simulink model "AXU5EV_R5_Reference"  (R2026b)
settings: Solver=FixedStepDiscrete  StopTime=0.1  FixedStep=Ts_ACR
undefined symbols (not defined in the file): Hold_Ticks, Id_Init_Step, Id_Init_Target, Id_Release_Ramp_Ticks, Iq_fric_run, Iq_fric_start, Iq_int_limit, Kaw_d, Kaw_q, Kaw_s, Ki_ACR, Ki_ASR, Kp_ACR, Kp_ASR, Kp_pos, PMLSM_Ld_H, PMLSM_Lq_H, PMLSM_psi_f_Wb, Pos_deadband, Ramp_Ticks, Speed_loop_Iq_Limit, T_pwm, Tau_e_mm, theta_align_const, Ts, Ts_ACR, Ts_ASR, Udc, v_ff_eps, v_over_eps, V_pos_max_mmps, v_ref_max, v_ref_set_step_dn, v_ref_set_step_up, v_ref_zero_eps, v_stick_off, v_stick_on
libraries: simulink x7, mcbeeMathTransformLib x2
settings Model: Creator=lww  LastModifiedBy=lww
settings OptimizationCC: DefaultParameterBehavior=Inlined  DifferentSizesBufferReuse=on  EfficientTunableParamExpr=on  EnhancedBackFolding=on  OptimizationCustomize=off  OptimizeBlockOrder=speed  PassReuseOutputArgsAs=Individual arguments  RemoveInternalMemoryZeroInit=on  RemoveRootLevelIOMemoryZeroInit=on
settings DebuggingCC: ParameterTunabilityLossMsg=error
settings SFSimCC: MATLABDynamicMemAlloc=off
settings RTWCC: DataTypeReplacement=CDataTypesFixedWidth  Description=Embedded Coder  GenCodeOnly=on  SystemTargetFile=ert.tlc  TemplateMakefile=ert_default_tmf
settings CodeAppCC: ForceParamTrailComments=on  IgnoreCustomStorageClasses=off  InsertBlockDesc=on  OperatorAnnotations=on  SFDataObjDesc=on  SimulinkDataObjDesc=on
settings ERTTargetCC: CombineSignalStateStructs=on  GenerateSampleERTMain=on  MaxIdInt16=INT16_MAX  MaxIdInt32=INT32_MAX  MaxIdInt64=INT64_MAX  MaxIdInt8=INT8_MAX  MaxIdUint16=UINT16_MAX  MaxIdUint32=UINT32_MAX  MaxIdUint64=UINT64_MAX  MaxIdUint8=UINT8_MAX  MinIdInt16=INT16_MIN  MinIdInt32=INT32_MIN  MinIdInt64=INT64_MIN  MinIdInt8=INT8_MIN

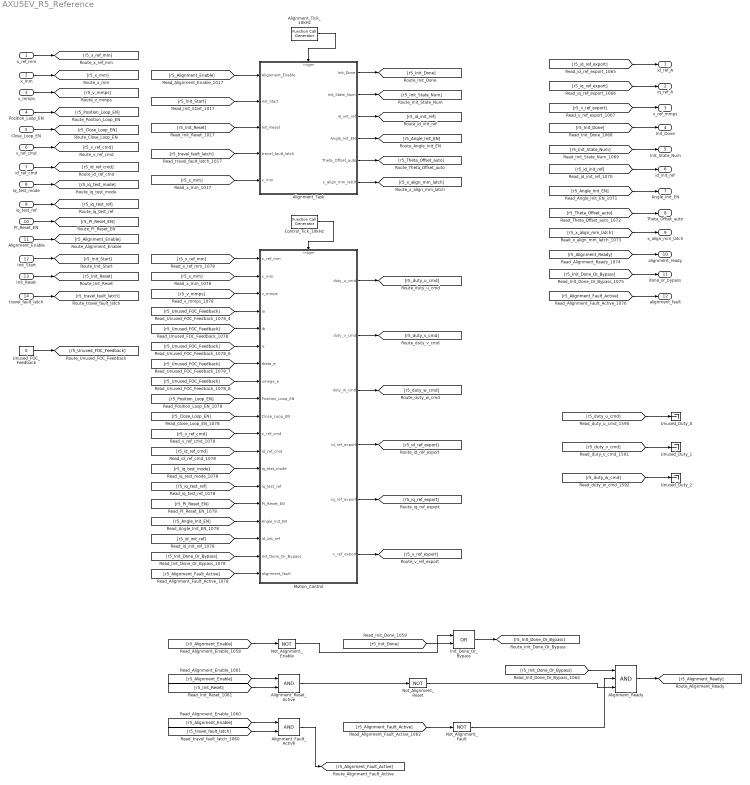
== system AXU5EV_R5_Reference ==
  x_ref_mm : Inport  OutDataTypeStr=double  SampleTime=Ts_ACR
  x_mm : Inport  Port=2  OutDataTypeStr=double  SampleTime=Ts_ACR
  v_mmps : Inport  Port=3  OutDataTypeStr=double  SampleTime=Ts_ACR
  Position_Loop_EN : Inport  Port=4  OutDataTypeStr=double  SampleTime=Ts_ACR
  Close_Loop_EN : Inport  Port=5  OutDataTypeStr=double  SampleTime=Ts_ACR
  v_ref_cmd : Inport  Port=6  OutDataTypeStr=double  SampleTime=Ts_ACR
  id_ref_cmd : Inport  Port=7  OutDataTypeStr=double  SampleTime=Ts_ACR
  iq_test_mode : Inport  Port=8  OutDataTypeStr=double  SampleTime=Ts_ACR
  iq_test_ref : Inport  Port=9  OutDataTypeStr=double  SampleTime=Ts_ACR
  PI_Reset_EN : Inport  Port=10  OutDataTypeStr=double  SampleTime=Ts_ACR
  Alignment_Enable : Inport  Port=11  OutDataTypeStr=double  SampleTime=Ts_ACR
  Init_Start : Inport  Port=12  OutDataTypeStr=double  SampleTime=Ts_ACR
  Init_Reset : Inport  Port=13  OutDataTypeStr=double  SampleTime=Ts_ACR
  travel_fault_latch : Inport  Port=14  OutDataTypeStr=double  SampleTime=Ts_ACR
  Alignment_Fault_Active : Logic  IconShape=distinctive  AllPortsSameDT=off  OutDataTypeStr=boolean
  Alignment_Ready : Logic  Inputs=3  IconShape=distinctive  AllPortsSameDT=off  OutDataTypeStr=boolean
  Alignment_Reset_Active : Logic  IconShape=distinctive  AllPortsSameDT=off  OutDataTypeStr=boolean
  Alignment_Task : Subsystem
  Alignment_Tick_10kHz : FunctionCallGenerator  Priority=-100  SampleTime=Ts
  Control_Tick_10kHz : FunctionCallGenerator  Priority=100  SampleTime=Ts
  Init_Done_Or_Bypass : Logic  Operator=OR  IconShape=distinctive  AllPortsSameDT=off  OutDataTypeStr=boolean
  Motion_Control : Subsystem
  Not_Alignment_Enable : Logic  Operator=NOT  IconShape=distinctive  AllPortsSameDT=off  OutDataTypeStr=boolean
  Not_Alignment_Fault : Logic  Operator=NOT  IconShape=distinctive  AllPortsSameDT=off  OutDataTypeStr=boolean
  Not_Alignment_Reset : Logic  Operator=NOT  IconShape=distinctive  AllPortsSameDT=off  OutDataTypeStr=boolean
  Unused_Duty_0 : Terminator
  Unused_Duty_1 : Terminator
  Unused_Duty_2 : Terminator
  Unused_FOC_Feedback : Constant  Value=0
  id_ref_A : Outport
  iq_ref_A : Outport  Port=2
  v_ref_mmps : Outport  Port=3
  Init_Done : Outport  Port=4
  Init_State_Num : Outport  Port=5
  id_init_ref : Outport  Port=6
  Angle_Init_EN : Outport  Port=7
  Theta_Offset_auto : Outport  Port=8
  x_align_mm_latch : Outport  Port=9
  alignment_ready : Outport  Port=10
  done_or_bypass : Outport  Port=11
  alignment_fault : Outport  Port=12
  wires:
  Unused_FOC_Feedback/1 -> [r5_Unused_FOC_Feedback]
  [r5_Unused_FOC_Feedback] -> Motion_Control/5(ib)
  Alignment_Ready/1 -> [r5_Alignment_Ready]
  [r5_Alignment_Ready] -> alignment_ready/1
  Alignment_Fault_Active/1 -> [r5_Alignment_Fault_Active]
  [r5_Alignment_Fault_Active] -> Not_Alignment_Fault/1
  [r5_Alignment_Fault_Active] -> alignment_fault/1
  [r5_Alignment_Fault_Active] -> Motion_Control/19(alignment_fault)
  Init_Done_Or_Bypass/1 -> [r5_Init_Done_Or_Bypass]
  [r5_Init_Done_Or_Bypass] -> Motion_Control/18(Init_Done_Or_Bypass)
  [r5_Init_Done_Or_Bypass] -> done_or_bypass/1
  [r5_Init_Done_Or_Bypass] -> Alignment_Ready/1
  Motion_Control/6(v_ref_export) -> [r5_v_ref_export]
  [r5_v_ref_export] -> v_ref_mmps/1
  Motion_Control/5(iq_ref_export) -> [r5_iq_ref_export]
  [r5_iq_ref_export] -> iq_ref_A/1
  Motion_Control/4(id_ref_export) -> [r5_id_ref_export]
  [r5_id_ref_export] -> id_ref_A/1
  Motion_Control/3(duty_w_cmd) -> [r5_duty_w_cmd]
  [r5_duty_w_cmd] -> Unused_Duty_2/1
  Motion_Control/2(duty_v_cmd) -> [r5_duty_v_cmd]
  [r5_duty_v_cmd] -> Unused_Duty_1/1
  Motion_Control/1(duty_u_cmd) -> [r5_duty_u_cmd]
  [r5_duty_u_cmd] -> Unused_Duty_0/1
  Alignment_Task/6(x_align_mm_latch) -> [r5_x_align_mm_latch]
  [r5_x_align_mm_latch] -> x_align_mm_latch/1
  Alignment_Task/5(Theta_Offset_auto) -> [r5_Theta_Offset_auto]
  [r5_Theta_Offset_auto] -> Theta_Offset_auto/1
  Alignment_Task/4(Angle_Init_EN) -> [r5_Angle_Init_EN]
  [r5_Angle_Init_EN] -> Angle_Init_EN/1
  [r5_Angle_Init_EN] -> Motion_Control/16(Angle_Init_EN)
  Alignment_Task/3(id_init_ref) -> [r5_id_init_ref]
  [r5_id_init_ref] -> id_init_ref/1
  [r5_id_init_ref] -> Motion_Control/17(id_init_ref)
  Alignment_Task/2(Init_State_Num) -> [r5_Init_State_Num]
  [r5_Init_State_Num] -> Init_State_Num/1
  Alignment_Task/1(Init_Done) -> [r5_Init_Done]
  [r5_Init_Done] -> Init_Done_Or_Bypass/2
  [r5_Init_Done] -> Init_Done/1
  travel_fault_latch/1 -> [r5_travel_fault_latch]
  [r5_travel_fault_latch] -> Alignment_Fault_Active/2
  [r5_travel_fault_latch] -> Alignment_Task/4(travel_fault_latch)
  Init_Reset/1 -> [r5_Init_Reset]
  [r5_Init_Reset] -> Alignment_Task/3(Init_Reset)
  [r5_Init_Reset] -> Alignment_Reset_Active/2
  Init_Start/1 -> [r5_Init_Start]
  [r5_Init_Start] -> Alignment_Task/2(Init_Start)
  Alignment_Enable/1 -> [r5_Alignment_Enable]
  [r5_Alignment_Enable] -> Alignment_Fault_Active/1
  [r5_Alignment_Enable] -> Not_Alignment_Enable/1
  [r5_Alignment_Enable] -> Alignment_Reset_Active/1
  [r5_Alignment_Enable] -> Alignment_Task/1(Alignment_Enable)
  PI_Reset_EN/1 -> [r5_PI_Reset_EN]
  [r5_PI_Reset_EN] -> Motion_Control/15(PI_Reset_EN)
  iq_test_ref/1 -> [r5_iq_test_ref]
  [r5_iq_test_ref] -> Motion_Control/14(iq_test_ref)
  iq_test_mode/1 -> [r5_iq_test_mode]
  [r5_iq_test_mode] -> Motion_Control/13(iq_test_mode)
  id_ref_cmd/1 -> [r5_id_ref_cmd]
  [r5_id_ref_cmd] -> Motion_Control/12(id_ref_cmd)
  v_ref_cmd/1 -> [r5_v_ref_cmd]
  [r5_v_ref_cmd] -> Motion_Control/11(v_ref_cmd)
  Close_Loop_EN/1 -> [r5_Close_Loop_EN]
  [r5_Close_Loop_EN] -> Motion_Control/10(Close_Loop_EN)
  Position_Loop_EN/1 -> [r5_Position_Loop_EN]
  [r5_Position_Loop_EN] -> Motion_Control/9(Position_Loop_EN)
  v_mmps/1 -> [r5_v_mmps]
  [r5_v_mmps] -> Motion_Control/3(v_mmps)
  x_mm/1 -> [r5_x_mm]
  [r5_x_mm] -> Motion_Control/2(x_mm)
  [r5_x_mm] -> Alignment_Task/5(x_mm)
  x_ref_mm/1 -> [r5_x_ref_mm]
  [r5_x_ref_mm] -> Motion_Control/1(x_ref_mm)
  Not_Alignment_Fault/1 -> Alignment_Ready/2
  Alignment_Tick_10kHz/1 -> Alignment_Task/Trigger
  Control_Tick_10kHz/1 -> Motion_Control/Trigger
  Alignment_Reset_Active/1 -> Not_Alignment_Reset/1
  Not_Alignment_Enable/1 -> Init_Done_Or_Bypass/1
  Not_Alignment_Reset/1 -> Alignment_Ready/3
  [r5_Unused_FOC_Feedback] -> Motion_Control/8(omega_e)
  [r5_Unused_FOC_Feedback] -> Motion_Control/7(theta_e)
  [r5_Unused_FOC_Feedback] -> Motion_Control/6(ic)
  [r5_Unused_FOC_Feedback] -> Motion_Control/4(ia)

== system AXU5EV_R5_Reference/Alignment_Task ==
  Alignment_Enable : Inport
  Init_Start : Inport  Port=2
  Init_Reset : Inport  Port=3
  travel_fault_latch : Inport  Port=4
  x_mm : Inport  Port=5
  Tick : TriggerPort  TriggerType=function-call  VariantControl=(inherit)
  Enabled_Original_MIL : Subsystem
  Init_Done : Outport
  Init_State_Num : Outport  Port=2
  id_init_ref : Outport  Port=3
  Angle_Init_EN : Outport  Port=4
  Theta_Offset_auto : Outport  Port=5
  x_align_mm_latch : Outport  Port=6
  wires:
  Enabled_Original_MIL/6(x_align_mm_latch) -> x_align_mm_latch/1
  Enabled_Original_MIL/5(Theta_Offset_auto) -> Theta_Offset_auto/1
  Enabled_Original_MIL/4(Angle_Init_EN) -> Angle_Init_EN/1
  Enabled_Original_MIL/1(Init_Done) -> Init_Done/1
  x_mm/1 -> Enabled_Original_MIL/4(x_mm)
  travel_fault_latch/1 -> Enabled_Original_MIL/3(travel_fault_latch)
  Init_Reset/1 -> Enabled_Original_MIL/2(Init_Reset)
  Enabled_Original_MIL/3(id_init_ref) -> id_init_ref/1
  Init_Start/1 -> Enabled_Original_MIL/1(Init_Start)
  Enabled_Original_MIL/2(Init_State_Num) -> Init_State_Num/1
  Alignment_Enable/1 -> Enabled_Original_MIL/Enable

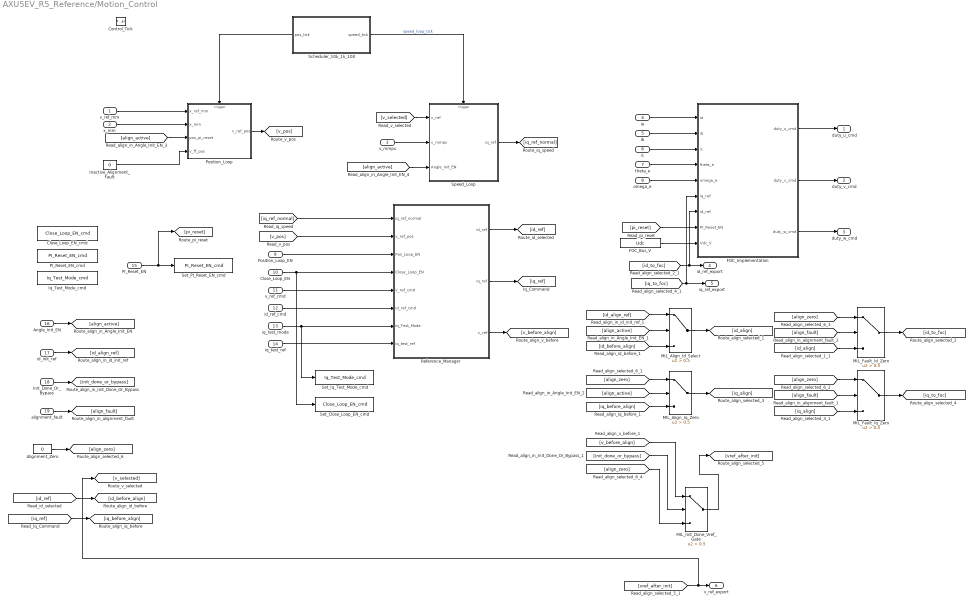
== system AXU5EV_R5_Reference/Motion_Control ==
  x_ref_mm : Inport
  x_mm : Inport  Port=2
  v_mmps : Inport  Port=3
  ia : Inport  Port=4
  ib : Inport  Port=5
  ic : Inport  Port=6
  theta_e : Inport  Port=7
  omega_e : Inport  Port=8
  Position_Loop_EN : Inport  Port=9
  Close_Loop_EN : Inport  Port=10
  v_ref_cmd : Inport  Port=11
  id_ref_cmd : Inport  Port=12
  iq_test_mode : Inport  Port=13
  iq_test_ref : Inport  Port=14
  PI_Reset_EN : Inport  Port=15
  Angle_Init_EN : Inport  Port=16
  id_init_ref : Inport  Port=17
  Init_Done_Or_Bypass : Inport  Port=18
  alignment_fault : Inport  Port=19
  Control_Tick : TriggerPort  TriggerType=function-call  VariantControl=(inherit)  PortDimensions=1
  Alignment_Zero : Constant  Value=0
  Close_Loop_EN_cmd : DataStoreMemory  DataStoreName=Close_Loop_EN_cmd  WriteAfterWriteMsg=warning  InitialValue=1  ShowAdditionalParam=off
  FOC_Bus_V : Constant  Value=Udc  SampleTime=-1
  FOC_Implementation : Subsystem  Variant=on  EmptyChoice=on
  Inactive_Alignment_Fault : Constant  Value=0
  Iq_Test_Mode_cmd : DataStoreMemory  DataStoreName=Iq_Test_Mode_cmd  WriteAfterWriteMsg=warning  ShowAdditionalParam=off
  MIL_Align_Id_Select : Switch  Criteria=u2 > Threshold  Threshold=0.5  SaturateOnIntegerOverflow=off  InputSameDT=off
  MIL_Align_Iq_Zero : Switch  Criteria=u2 > Threshold  Threshold=0.5  SaturateOnIntegerOverflow=off  InputSameDT=off
  MIL_Fault_Id_Zero : Switch  Criteria=u2 > Threshold  Threshold=0.5  SaturateOnIntegerOverflow=off  InputSameDT=off
  MIL_Fault_Iq_Zero : Switch  Criteria=u2 > Threshold  Threshold=0.5  SaturateOnIntegerOverflow=off  InputSameDT=off
  MIL_Init_Done_Vref_Gate : Switch  Criteria=u2 > Threshold  Threshold=0.5  SaturateOnIntegerOverflow=off  InputSameDT=off
  PI_Reset_EN_cmd : DataStoreMemory  DataStoreName=PI_Reset_EN_cmd  WriteAfterWriteMsg=warning  ShowAdditionalParam=off
  Position_Loop : Subsystem  TreatAsAtomicUnit=on
  Reference_Manager : Subsystem
  Scheduler_10k_1k_100 : Subsystem
      settings: PortSchema="{\"entries\":[{\"content\":{\"sides\":[{\"content\":{\"connectorIds\":[\"Out2\"]},\"type\":\"ConnectorPlacement.EquallySpacedRectSide\",\"uuid\":\"7a2cd2ad-1b6d-4ced-b4c0-dea2e76e4441\"},{\"content\":{\"connectorIds\":[\"Out1\"],\"side\":\"RIGHT\"},\"type\":\"ConnectorPlacement.EquallySpacedRectSide\",\"uuid\":\"f7db3b94-1126-4089-83bd-8e57d20e6fd7\"},{\"content\":{\"side\":\"TOP\"},\"type\":\"ConnectorPlacement.EquallySpacedRectSide\",\"uuid\":\"9153f6b5-22af-48be-92c0-68be43f93648\"}]},\"type\":\"ConnectorPlacement.EquallySpacedConnector\",\"uuid\":\"029fb485-bddc-4cd2-9c64-7547c8dffd2b\"}],\"packageUris\":[\"http://schema.mathworks.com/mf0/Connector/R2020b\"],\"version\":\"1.0\"}"
  Set_Close_Loop_EN_cmd : DataStoreWrite  Priority=-10  DataStoreName=Close_Loop_EN_cmd  IndexOptions=Index vector (dialog)  Indices=1  OutputSizes=1
  Set_Iq_Test_Mode_cmd : DataStoreWrite  Priority=-10  DataStoreName=Iq_Test_Mode_cmd  IndexOptions=Index vector (dialog)  Indices=1  OutputSizes=1
  Set_PI_Reset_EN_cmd : DataStoreWrite  Priority=-10  DataStoreName=PI_Reset_EN_cmd  IndexOptions=Index vector (dialog)  Indices=1  OutputSizes=1
  Speed_Loop : Subsystem  TreatAsAtomicUnit=on
  duty_u_cmd : Outport
  duty_v_cmd : Outport  Port=2
  duty_w_cmd : Outport  Port=3
  id_ref_export : Outport  Port=4
  iq_ref_export : Outport  Port=5
  v_ref_export : Outport  Port=6
  wires:
  FOC_Bus_V/1 -> FOC_Implementation/9(Vdc_V)
  FOC_Implementation/3(duty_w_cmd) -> duty_w_cmd/1
  FOC_Implementation/2(duty_v_cmd) -> duty_v_cmd/1
  FOC_Implementation/1(duty_u_cmd) -> duty_u_cmd/1
  [pi_reset] -> FOC_Implementation/8(PI_Reset_EN)
  omega_e/1 -> FOC_Implementation/5(omega_e)
  theta_e/1 -> FOC_Implementation/4(theta_e)
  ic/1 -> FOC_Implementation/3(ic)
  ib/1 -> FOC_Implementation/2(ib)
  ia/1 -> FOC_Implementation/1(ia)
  Reference_Manager/3(v_ref) -> [v_before_align]
  [iq_before_align] -> MIL_Align_Iq_Zero/3
  [iq_ref] -> [iq_before_align]
  [id_before_align] -> MIL_Align_Id_Select/3
  [id_ref] -> [id_before_align]
  [align_fault] -> MIL_Fault_Id_Zero/2
  [align_fault] -> MIL_Fault_Iq_Zero/2
  alignment_fault/1 -> [align_fault]
  Init_Done_Or_Bypass/1 -> [init_done_or_bypass]
  [id_align_ref] -> MIL_Align_Id_Select/1
  id_init_ref/1 -> [id_align_ref]
  [align_active] -> Speed_Loop/3(Angle_Init_EN)
  [align_active] -> Position_Loop/3(pos_pi_reset)
  [align_active] -> MIL_Align_Iq_Zero/2
  [align_active] -> MIL_Align_Id_Select/2
  Angle_Init_EN/1 -> [align_active]
  [align_zero] -> MIL_Fault_Id_Zero/1
  [align_zero] -> MIL_Fault_Iq_Zero/1
  [align_zero] -> MIL_Align_Iq_Zero/1
  Alignment_Zero/1 -> [align_zero]
  MIL_Fault_Iq_Zero/1 -> [iq_to_foc]
  [iq_align] -> MIL_Fault_Iq_Zero/3
  MIL_Align_Iq_Zero/1 -> [iq_align]
  MIL_Fault_Id_Zero/1 -> [id_to_foc]
  [id_align] -> MIL_Fault_Id_Zero/3
  MIL_Align_Id_Select/1 -> [id_align]
  Reference_Manager/2(iq_ref) -> [iq_ref]
  Reference_Manager/1(id_ref) -> [id_ref]
  v_mmps/1 -> Speed_Loop/2(v_mmps)
  Close_Loop_EN/1 -> Reference_Manager/4(Close_Loop_EN), Set_Close_Loop_EN_cmd/1
  iq_test_mode/1 -> Reference_Manager/7(Iq_Test_Mode), Set_Iq_Test_Mode_cmd/1
  PI_Reset_EN/1 -> Set_PI_Reset_EN_cmd/1, [pi_reset]
  Scheduler_10k_1k_100/2(pos_tick) -> Position_Loop/Trigger
  Scheduler_10k_1k_100/1(speed_tick) -> Speed_Loop/Trigger  "speed_loop_tick"
  x_ref_mm/1 -> Position_Loop/1(x_ref_mm)
  x_mm/1 -> Position_Loop/2(x_mm)
  Position_Loop/1(v_ref_pos) -> [v_pos]
  Speed_Loop/1(iq_ref) -> [iq_ref_normal]
  Inactive_Alignment_Fault/1 -> Position_Loop/4(v_ff_pos)
  [v_pos] -> Reference_Manager/2(v_ref_pos)
  [iq_ref_normal] -> Reference_Manager/1(iq_ref_normal)
  [v_selected] -> Speed_Loop/1(v_ref)
  Position_Loop_EN/1 -> Reference_Manager/3(Pos_Loop_EN)
  v_ref_cmd/1 -> Reference_Manager/5(v_ref_cmd)
  id_ref_cmd/1 -> Reference_Manager/6(id_ref_cmd)
  iq_test_ref/1 -> Reference_Manager/8(iq_test_ref)
  MIL_Init_Done_Vref_Gate/1 -> [vref_after_init]
  [vref_after_init] -> v_ref_export/1, [v_selected]
  [align_zero] -> MIL_Init_Done_Vref_Gate/3
  [init_done_or_bypass] -> MIL_Init_Done_Vref_Gate/2
  [v_before_align] -> MIL_Init_Done_Vref_Gate/1
  [iq_to_foc] -> iq_ref_export/1, FOC_Implementation/6(iq_ref)
  [id_to_foc] -> id_ref_export/1, FOC_Implementation/7(id_ref)

== system AXU5EV_R5_Reference/Alignment_Task/Enabled_Original_MIL ==
  Init_Start : Inport
  Init_Reset : Inport  Port=2
  travel_fault_latch : Inport  Port=3
  x_mm : Inport  Port=4
  Enable : EnablePort
  Angle_Init : Stateflow chart  TreatAsAtomicUnit=on
  Init_Done : Outport
  Init_State_Num : Outport  Port=2
  id_init_ref : Outport  Port=3
  Angle_Init_EN : Outport  Port=4
  Theta_Offset_auto : Outport  Port=5
  x_align_mm_latch : Outport  Port=6
  wires:
  Angle_Init/4(Angle_Init_EN) -> Angle_Init_EN/1  "Angle_Init_EN"
  Angle_Init/5(Theta_Offset_auto) -> Theta_Offset_auto/1  "Theta_Offset_auto"
  Angle_Init/6(x_align_mm_latch) -> x_align_mm_latch/1  "x_align_mm_latch"
  Angle_Init/3(id_init_ref) -> id_init_ref/1  "id_init_ref"
  Angle_Init/2(Init_State_Num) -> Init_State_Num/1  "Init_State_Num"
  Angle_Init/1(Init_Done) -> Init_Done/1  "Init_Done"
  x_mm/1 -> Angle_Init/4(x_mm)
  travel_fault_latch/1 -> Angle_Init/3(travel_fault_latch)
  Init_Reset/1 -> Angle_Init/2(Init_Reset)
  Init_Start/1 -> Angle_Init/1(Init_Start)

== system AXU5EV_R5_Reference/Motion_Control/FOC_Implementation ==
  ia : Inport
  ib : Inport  Port=2
  ic : Inport  Port=3
  theta_e : Inport  Port=4
  omega_e : Inport  Port=5
  iq_ref : Inport  Port=6
  id_ref : Inport  Port=7
  PI_Reset_EN : Inport  Port=8
  Vdc_V : Inport  Port=9
  Fixed : Subsystem  VariantControl=FOC_Impl_Select == 1
  Float : Subsystem  VariantControl=FOC_Impl_Select == 0
  duty_u_cmd : Outport
  duty_v_cmd : Outport  Port=2
  duty_w_cmd : Outport  Port=3

== system AXU5EV_R5_Reference/Motion_Control/Position_Loop ==
  x_ref_mm : Inport
  x_mm : Inport  Port=2
  pos_pi_reset : Inport  Port=3
  v_ff_pos : Inport  Port=4
  Trigger : TriggerPort  VariantControl=(inherit)
  Dead Zone : DeadZone  LowerValue=-Pos_deadband  UpperValue=+Pos_deadband
  Gain : Gain  Gain=Kp_pos
  Saturation : Saturate  UpperLimit=V_pos_max_mmps  LowerLimit=-V_pos_max_mmps
  Sum : Sum  Inputs=|+-
  Sum1 : Sum  Inputs=|++
  Terminator : Terminator
  v_ref_pos : Outport
  wires:
  Saturation/1 -> v_ref_pos/1  "obs_v_ref_pos"
  pos_pi_reset/1 -> Terminator/1
  Sum1/1 -> Saturation/1
  v_ff_pos/1 -> Sum1/2
  Gain/1 -> Sum1/1
  Dead Zone/1 -> Gain/1
  Sum/1 -> Dead Zone/1  "e_pos"
  x_mm/1 -> Sum/2
  x_ref_mm/1 -> Sum/1

== system AXU5EV_R5_Reference/Motion_Control/Reference_Manager ==
  iq_ref_normal : Inport
  v_ref_pos : Inport  Port=2
  Pos_Loop_EN : Inport  Port=3
  Close_Loop_EN : Inport  Port=4
  v_ref_cmd : Inport  Port=5
  id_ref_cmd : Inport  Port=6
  Iq_Test_Mode : Inport  Port=7
  iq_test_ref : Inport  Port=8
  Constant15 : Constant  Value=0
  Saturation : Saturate  UpperLimit=v_ref_max  LowerLimit=-v_ref_max
  Switch : Switch  Criteria=u2 > Threshold  Threshold=0.5  SaturateOnIntegerOverflow=off  InputSameDT=off
  Switch9 : Switch  Criteria=u2 > Threshold  Threshold=0.5  SaturateOnIntegerOverflow=off  InputSameDT=off
  v_ref_closed_sel : Switch  Criteria=u2 > Threshold  Threshold=0.5  SaturateOnIntegerOverflow=off  InputSameDT=off
  v_ref_set_slew_limiter : Subsystem
  id_ref : Outport
  iq_ref : Outport  Port=2
  v_ref : Outport  Port=3
  wires:
  v_ref_cmd/1 -> v_ref_closed_sel/3
  Saturation/1 -> Switch9/1
  Pos_Loop_EN/1 -> v_ref_closed_sel/2
  v_ref_closed_sel/1 -> v_ref_set_slew_limiter/1(v_ref_set)  "v_ref_closed"
  v_ref_pos/1 -> v_ref_closed_sel/1
  v_ref_set_slew_limiter/1(v_ref_set_limited) -> Saturation/1
  id_ref_cmd/1 -> id_ref/1
  iq_ref_normal/1 -> Switch/3
  Constant15/1 -> Switch9/3
  Iq_Test_Mode/1 -> Switch/2
  iq_test_ref/1 -> Switch/1
  Close_Loop_EN/1 -> Switch9/2
  Switch9/1 -> v_ref/1
  Switch/1 -> iq_ref/1

== system AXU5EV_R5_Reference/Motion_Control/Scheduler_10k_1k_100 ==
  note: speed 计数链(/10)
  note: position 计数链(/100)
  Add1 : Sum
  Add2 : Sum
  Constant1 : Constant
  Constant2 : Constant  Value=0
  Constant3 : Constant
  Constant4 : Constant  Value=0
  Logical Operator : Logic  AllPortsSameDT=off  OutDataTypeStr=boolean
  pos_cnt_hold_sel : Switch  Criteria=u2 > Threshold  Threshold=0.5  SaturateOnIntegerOverflow=off  InputSameDT=off
  pos_cnt_update_sel : Switch  Criteria=u2 > Threshold  Threshold=0.5  SaturateOnIntegerOverflow=off  InputSameDT=off
  pos_cnt_z : UnitDelay  SampleTime=-1
  pos_tc : simulink/Logic and Bit Operations/Compare To Constant  relop=>=  const=10  OutDataTypeStr=boolean
  spd_cnt_next_sel : Switch  Criteria=u2 > Threshold  Threshold=0.5  SaturateOnIntegerOverflow=off  InputSameDT=off
  spd_cnt_z : UnitDelay  SampleTime=-1
  spd_tc : simulink/Logic and Bit Operations/Compare To Constant  relop=>=  const=10  OutDataTypeStr=boolean
  speed_tick : Outport
  pos_tick : Outport  Port=2
  wires:
  Logical Operator/1 -> pos_tick/1
  pos_cnt_hold_sel/1 -> pos_cnt_z/1
  pos_cnt_update_sel/1 -> pos_cnt_hold_sel/1  "pos_cnt_update_candidate"
  Constant4/1 -> pos_cnt_update_sel/1
  pos_tc/1 -> pos_cnt_update_sel/2, Logical Operator/2
  Add2/1 -> pos_tc/1, pos_cnt_update_sel/3  "pos_cnt_inc"
  Constant3/1 -> Add2/2
  pos_cnt_z/1 -> pos_cnt_hold_sel/3, Add2/1
  Add1/1 -> spd_tc/1, spd_cnt_next_sel/3  "spd_cnt_inc"
  spd_cnt_next_sel/1 -> spd_cnt_z/1
  Constant2/1 -> spd_cnt_next_sel/1
  Constant1/1 -> Add1/2
  spd_tc/1 -> spd_cnt_next_sel/2, pos_cnt_hold_sel/2, Logical Operator/1, speed_tick/1
  spd_cnt_z/1 -> Add1/1

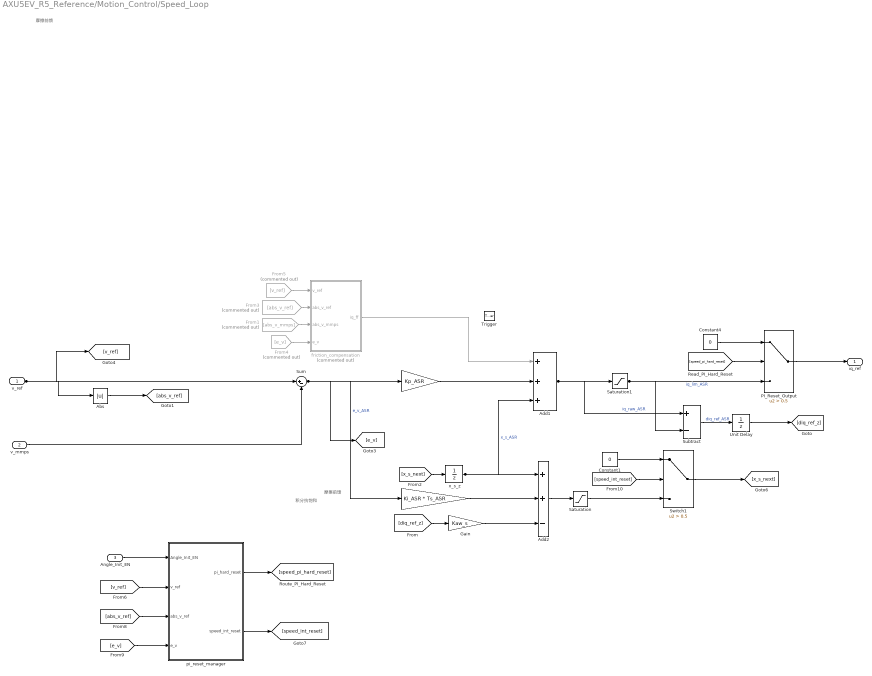
== system AXU5EV_R5_Reference/Motion_Control/Speed_Loop ==
  note: 摩擦前馈
  note: 积分抗饱和
  note: 摩擦前馈
  v_ref : Inport
  v_mmps : Inport  Port=2
  Angle_Init_EN : Inport  Port=3
  Trigger : TriggerPort  VariantControl=(inherit)
  " " : Gain  Gain=Ki_ASR * Ts_ASR
  "  " : Gain  Gain=Kp_ASR
  Abs : Abs  SaturateOnIntegerOverflow=off
  Add1 : Sum  Inputs=+++
  Add2 : Sum  Inputs=++-
  Constant1 : Constant  Value=0
  Constant4 : Constant  Value=0
  From1 : From  Commented=on  GotoTag=abs_v_mmps
  From3 : From  Commented=on  GotoTag=abs_v_ref
  From4 : From  Commented=on  GotoTag=e_v
  From5 : From  Commented=on  GotoTag=v_ref
  Gain : Gain  Gain=Kaw_s
  PI_Reset_Output : Switch  Criteria=u2 > Threshold  Threshold=0.5  SaturateOnIntegerOverflow=off  InputSameDT=off
  Saturation : Saturate  UpperLimit=Iq_int_limit  LowerLimit=-Iq_int_limit
  Saturation1 : Saturate  UpperLimit=Speed_loop_Iq_Limit  LowerLimit=-Speed_loop_Iq_Limit
  Subtract : Sum  Inputs=+-
  Sum : Sum  Inputs=|+-
  Switch1 : Switch  Criteria=u2 > Threshold  Threshold=0.5  SaturateOnIntegerOverflow=off  InputSameDT=off
  Unit Delay : UnitDelay  SampleTime=-1
  friction_compensation : Subsystem  Commented=on
  pi_reset_manager : Subsystem
  x_s_z : UnitDelay  SampleTime=-1
  iq_ref : Outport
  wires:
  v_mmps/1 -> Sum/2
  Saturation/1 -> Switch1/3
  Switch1/1 -> [x_s_next]
  [speed_int_reset] -> Switch1/2
  pi_reset_manager/1(pi_hard_reset) -> [speed_pi_hard_reset]
  pi_reset_manager/2(speed_int_reset) -> [speed_int_reset]
  [speed_pi_hard_reset] -> PI_Reset_Output/2
  [e_v] -> pi_reset_manager/4(e_v)
  [abs_v_ref] -> pi_reset_manager/3(abs_v_ref)
  [v_ref] -> pi_reset_manager/2(v_ref)
  From5/1 -> friction_compensation/1(v_ref)
  Angle_Init_EN/1 -> pi_reset_manager/1(Angle_Init_EN)
  Abs/1 -> [abs_v_ref]
  From3/1 -> friction_compensation/2(abs_v_ref)
  From1/1 -> friction_compensation/3(abs_v_mmps)
  From4/1 -> friction_compensation/4(e_v)
  x_s_z/1 -> Add2/1, Add1/3  "x_s_ASR"
  friction_compensation/1(iq_ff) -> Add1/1
  "  "/1 -> Add1/2
  Constant4/1 -> PI_Reset_Output/1
  PI_Reset_Output/1 -> iq_ref/1
  Constant1/1 -> Switch1/1
  [diq_ref_z] -> Gain/1
  Unit Delay/1 -> [diq_ref_z]
  Subtract/1 -> Unit Delay/1  "diq_ref_ASR"
  " "/1 -> Add2/2
  Gain/1 -> Add2/3
  Add2/1 -> Saturation/1
  [x_s_next] -> x_s_z/1
  Saturation1/1 -> Subtract/2, PI_Reset_Output/3  "iq_lim_ASR"
  v_ref/1 -> [v_ref], Abs/1, Sum/1
  Add1/1 -> Saturation1/1, Subtract/1  "iq_raw_ASR"
  Sum/1 -> "  "/1, " "/1, [e_v]  "e_v_ASR"

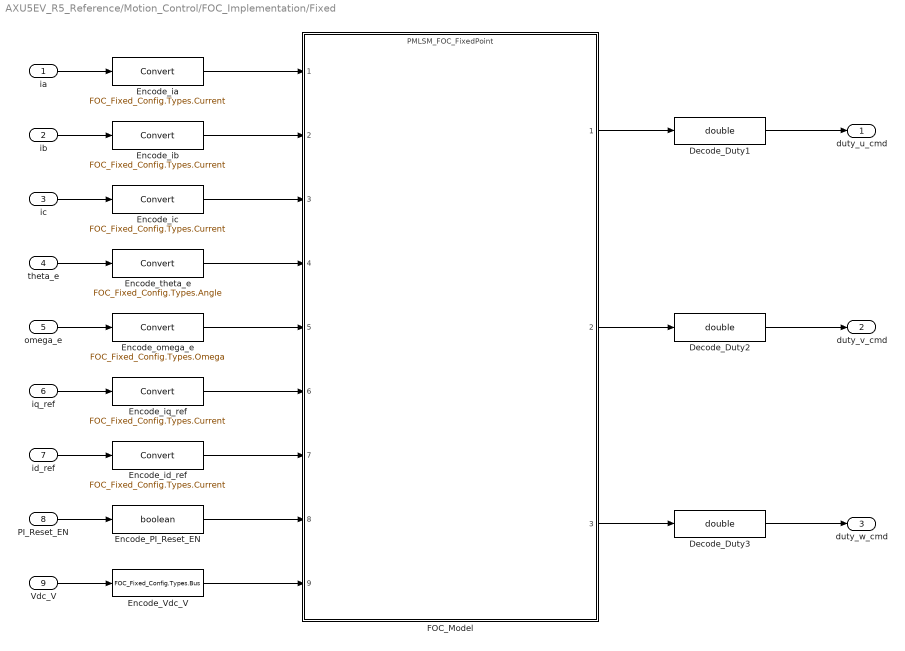
== system AXU5EV_R5_Reference/Motion_Control/FOC_Implementation/Fixed ==
  ia : Inport
  ib : Inport  Port=2
  ic : Inport  Port=3
  theta_e : Inport  Port=4
  omega_e : Inport  Port=5
  iq_ref : Inport  Port=6
  id_ref : Inport  Port=7
  PI_Reset_EN : Inport  Port=8
  Vdc_V : Inport  Port=9
  Decode_Duty1 : DataTypeConversion  OutDataTypeStr=double
  Decode_Duty2 : DataTypeConversion  OutDataTypeStr=double
  Decode_Duty3 : DataTypeConversion  OutDataTypeStr=double
  Encode_PI_Reset_EN : DataTypeConversion  OutDataTypeStr=boolean  RndMeth=Convergent
  Encode_Vdc_V : DataTypeConversion  OutDataTypeStr=FOC_Fixed_Config.Types.Bus  RndMeth=Convergent
  Encode_ia : DataTypeConversion  OutDataTypeStr=FOC_Fixed_Config.Types.Current  RndMeth=Convergent
  Encode_ib : DataTypeConversion  OutDataTypeStr=FOC_Fixed_Config.Types.Current  RndMeth=Convergent
  Encode_ic : DataTypeConversion  OutDataTypeStr=FOC_Fixed_Config.Types.Current  RndMeth=Convergent
  Encode_id_ref : DataTypeConversion  OutDataTypeStr=FOC_Fixed_Config.Types.Current  RndMeth=Convergent
  Encode_iq_ref : DataTypeConversion  OutDataTypeStr=FOC_Fixed_Config.Types.Current  RndMeth=Convergent
  Encode_omega_e : DataTypeConversion  OutDataTypeStr=FOC_Fixed_Config.Types.Omega  RndMeth=Convergent
  Encode_theta_e : DataTypeConversion  OutDataTypeStr=FOC_Fixed_Config.Types.Angle  RndMeth=Convergent
  FOC_Model : ModelReference  ModelNameDialog=PMLSM_FOC_FixedPoint  SimulationMode=Normal  ModelReferenceVersion=1.20
  duty_u_cmd : Outport
  duty_v_cmd : Outport  Port=2
  duty_w_cmd : Outport  Port=3
  wires:
  ia/1 -> Encode_ia/1
  ib/1 -> Encode_ib/1
  ic/1 -> Encode_ic/1
  theta_e/1 -> Encode_theta_e/1
  omega_e/1 -> Encode_omega_e/1
  Vdc_V/1 -> Encode_Vdc_V/1
  iq_ref/1 -> Encode_iq_ref/1
  id_ref/1 -> Encode_id_ref/1
  PI_Reset_EN/1 -> Encode_PI_Reset_EN/1
  Encode_ia/1 -> FOC_Model/1
  Encode_theta_e/1 -> FOC_Model/4
  Encode_ic/1 -> FOC_Model/3
  Encode_ib/1 -> FOC_Model/2
  Encode_PI_Reset_EN/1 -> FOC_Model/8
  Encode_id_ref/1 -> FOC_Model/7
  Encode_iq_ref/1 -> FOC_Model/6
  Encode_omega_e/1 -> FOC_Model/5
  Encode_Vdc_V/1 -> FOC_Model/9
  FOC_Model/1 -> Decode_Duty1/1
  FOC_Model/2 -> Decode_Duty2/1
  FOC_Model/3 -> Decode_Duty3/1
  Decode_Duty3/1 -> duty_w_cmd/1
  Decode_Duty2/1 -> duty_v_cmd/1
  Decode_Duty1/1 -> duty_u_cmd/1

== system AXU5EV_R5_Reference/Motion_Control/FOC_Implementation/Float ==
  ia : Inport
  ib : Inport  Port=2
  ic : Inport  Port=3
  theta_e : Inport  Port=4
  omega_e : Inport  Port=5
  iq_ref : Inport  Port=6
  id_ref : Inport  Port=7
  PI_Reset_EN : Inport  Port=8
  Vdc_V : Inport  Port=9
  FOC_Algorithm : Subsystem
  Original_Udc_Base_Reference : Terminator
  duty_u_cmd : Outport
  duty_v_cmd : Outport  Port=2
  duty_w_cmd : Outport  Port=3
  wires:
  Vdc_V/1 -> Original_Udc_Base_Reference/1
  PI_Reset_EN/1 -> FOC_Algorithm/8(PI_Reset_EN)
  id_ref/1 -> FOC_Algorithm/7(id_ref)
  FOC_Algorithm/2(duty_v_cmd) -> duty_v_cmd/1
  omega_e/1 -> FOC_Algorithm/5(omega_e)
  iq_ref/1 -> FOC_Algorithm/6(iq_ref)
  theta_e/1 -> FOC_Algorithm/4(theta_e)
  FOC_Algorithm/3(duty_w_cmd) -> duty_w_cmd/1
  FOC_Algorithm/1(duty_u_cmd) -> duty_u_cmd/1
  ib/1 -> FOC_Algorithm/2(ib)
  ic/1 -> FOC_Algorithm/3(ic)
  ia/1 -> FOC_Algorithm/1(ia)

== system AXU5EV_R5_Reference/Motion_Control/Reference_Manager/v_ref_set_slew_limiter ==
  v_ref_set : Inport
  Add : Sum
  Saturation : Saturate  UpperLimit=v_ref_set_step_up  LowerLimit=-v_ref_set_step_dn
  Subtract : Sum  Inputs=+-
  v_ref_set_lim_z : UnitDelay  SampleTime=-1
  v_ref_set_limited : Outport
  wires:
  Add/1 -> v_ref_set_lim_z/1, v_ref_set_limited/1
  Subtract/1 -> Saturation/1
  Saturation/1 -> Add/1
  v_ref_set/1 -> Subtract/1
  v_ref_set_lim_z/1 -> Subtract/2, Add/2

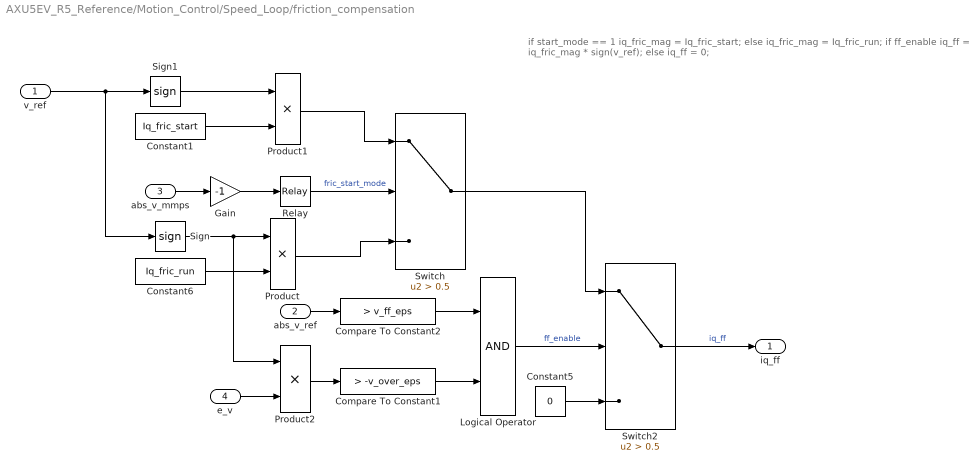
== system AXU5EV_R5_Reference/Motion_Control/Speed_Loop/friction_compensation ==
  note: if start_mode == 1
      | 	iq_fric_mag = Iq_fric_start;
      | else
      | 	iq_fric_mag = Iq_fric_run;
      |
      | if ff_enable
      | 	iq_ff = iq_fric_mag * sign(v_ref);
      |  else
      | 	iq_ff = 0;
  v_ref : Inport
  abs_v_ref : Inport  Port=2
  abs_v_mmps : Inport  Port=3
  e_v : Inport  Port=4
  Compare To Constant1 : simulink/Logic and Bit Operations/Compare To Constant  relop=>  const=-v_over_eps  OutDataTypeStr=boolean
  Compare To Constant2 : simulink/Logic and Bit Operations/Compare To Constant  relop=>  const=v_ff_eps  OutDataTypeStr=boolean
  Constant1 : Constant  Value=Iq_fric_start
  Constant5 : Constant  Value=0
  Constant6 : Constant  Value=Iq_fric_run
  Gain : Gain  Gain=-1
  Logical Operator : Logic  AllPortsSameDT=off  OutDataTypeStr=boolean
  Product : Product
  Product1 : Product
  Product2 : Product
  Relay : Relay  OnSwitchValue=-v_stick_on  OffSwitchValue=-v_stick_off
  Sign : Signum
  Sign1 : Signum
  Switch : Switch  Criteria=u2 > Threshold  Threshold=0.5  SaturateOnIntegerOverflow=off  InputSameDT=off
  Switch2 : Switch  Criteria=u2 > Threshold  Threshold=0.5  SaturateOnIntegerOverflow=off  InputSameDT=off
  iq_ff : Outport
  wires:
  Gain/1 -> Relay/1
  Relay/1 -> Switch/2  "fric_start_mode"
  abs_v_mmps/1 -> Gain/1
  Logical Operator/1 -> Switch2/2  "ff_enable"
  Compare To Constant1/1 -> Logical Operator/2
  Compare To Constant2/1 -> Logical Operator/1
  Product2/1 -> Compare To Constant1/1
  e_v/1 -> Product2/2
  Product1/1 -> Switch/1
  Constant1/1 -> Product1/2
  Sign1/1 -> Product1/1
  Product/1 -> Switch/3
  Switch/1 -> Switch2/1
  Switch2/1 -> iq_ff/1  "iq_ff"
  abs_v_ref/1 -> Compare To Constant2/1
  Constant6/1 -> Product/2
  Constant5/1 -> Switch2/3
  Sign/1 -> Product/1, Product2/1
  v_ref/1 -> Sign1/1, Sign/1

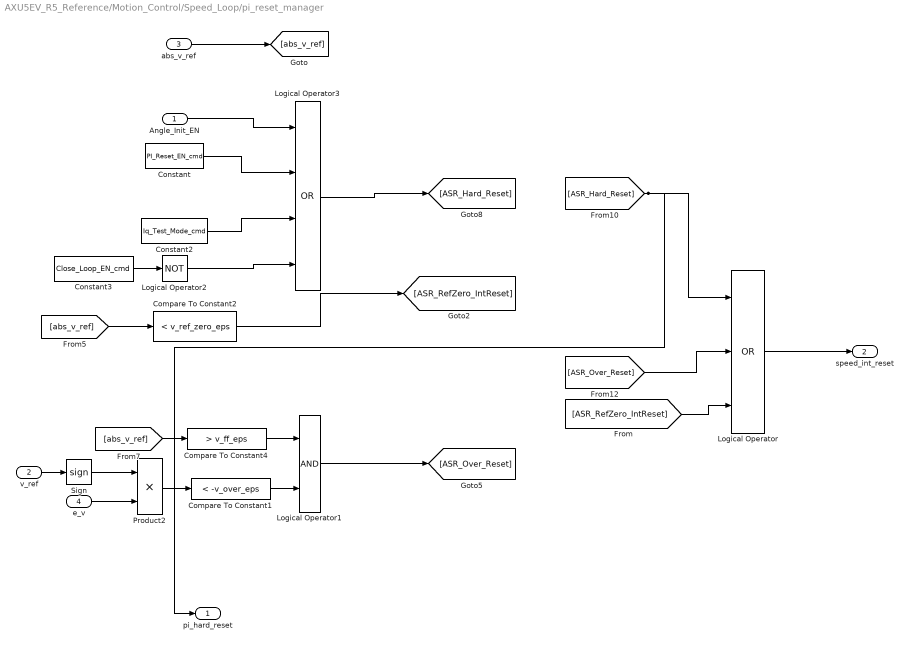
== system AXU5EV_R5_Reference/Motion_Control/Speed_Loop/pi_reset_manager ==
  Angle_Init_EN : Inport
  v_ref : Inport  Port=2
  abs_v_ref : Inport  Port=3
  e_v : Inport  Port=4
  Compare To Constant1 : simulink/Logic and Bit Operations/Compare To Constant  relop=<  const=-v_over_eps  OutDataTypeStr=boolean
  Compare To Constant2 : simulink/Logic and Bit Operations/Compare To Constant  relop=<  const=v_ref_zero_eps  OutDataTypeStr=boolean
  Compare To Constant4 : simulink/Logic and Bit Operations/Compare To Constant  relop=>  const=v_ff_eps  OutDataTypeStr=boolean
  Constant : DataStoreRead  DataStoreName=PI_Reset_EN_cmd  IndexOptions=Index vector (dialog)  Indices=1  OutputSizes=1
  Constant2 : DataStoreRead  DataStoreName=Iq_Test_Mode_cmd  IndexOptions=Index vector (dialog)  Indices=1  OutputSizes=1
  Constant3 : DataStoreRead  DataStoreName=Close_Loop_EN_cmd  IndexOptions=Index vector (dialog)  Indices=1  OutputSizes=1
  Logical Operator : Logic  Operator=OR  Inputs=3  AllPortsSameDT=off  OutDataTypeStr=boolean
  Logical Operator1 : Logic  AllPortsSameDT=off  OutDataTypeStr=boolean
  Logical Operator2 : Logic  Operator=NOT  AllPortsSameDT=off  OutDataTypeStr=boolean
  Logical Operator3 : Logic  Operator=OR  Inputs=4  AllPortsSameDT=off  OutDataTypeStr=boolean
  Product2 : Product
  Sign : Signum
  pi_hard_reset : Outport
  speed_int_reset : Outport  Port=2
  wires:
  Constant/1 -> Logical Operator3/2
  Constant3/1 -> Logical Operator2/1
  Constant2/1 -> Logical Operator3/3
  Logical Operator2/1 -> Logical Operator3/4
  Angle_Init_EN/1 -> Logical Operator3/1
  Logical Operator3/1 -> [ASR_Hard_Reset]
  [ASR_Hard_Reset] -> Logical Operator/1, pi_hard_reset/1
  [ASR_Over_Reset] -> Logical Operator/2
  Logical Operator/1 -> speed_int_reset/1
  [ASR_RefZero_IntReset] -> Logical Operator/3
  Logical Operator1/1 -> [ASR_Over_Reset]
  abs_v_ref/1 -> [abs_v_ref]
  v_ref/1 -> Sign/1
  Compare To Constant4/1 -> Logical Operator1/1
  Compare To Constant1/1 -> Logical Operator1/2
  Product2/1 -> Compare To Constant1/1
  Sign/1 -> Product2/1
  e_v/1 -> Product2/2
  [abs_v_ref] -> Compare To Constant4/1
  [abs_v_ref] -> Compare To Constant2/1
  Compare To Constant2/1 -> [ASR_RefZero_IntReset]

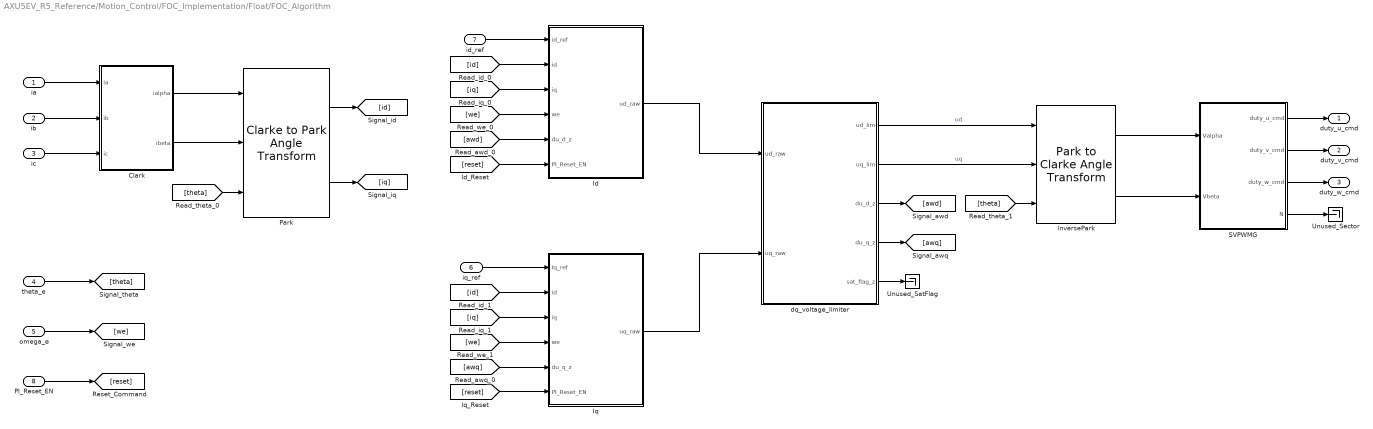
== system AXU5EV_R5_Reference/Motion_Control/FOC_Implementation/Float/FOC_Algorithm ==
  ia : Inport
  ib : Inport  Port=2
  ic : Inport  Port=3
  theta_e : Inport  Port=4
  omega_e : Inport  Port=5
  iq_ref : Inport  Port=6
  id_ref : Inport  Port=7
  PI_Reset_EN : Inport  Port=8
  Clark : Subsystem  TreatAsAtomicUnit=on  RTWFcnName=Clack_Fun
      settings: RTWFcnNameOpts=User specified
  Id : Subsystem  TreatAsAtomicUnit=on  RTWFcnName=Id_Fun
      settings: RTWFcnNameOpts=User specified
  InversePark : mcbeeMathTransformLib/Park to Clarke Angle Transform  AxisAlignment=D-axis  UseWithEmbedded=on  PhaseInput=Two inputs  ThetaInput=Electrical position  AngleInput=Radians  N_points=1024
      settings: LibrarySourceBlock=mcbhdllib/Controls/Math Transforms/Inverse Park Transform
  Iq : Subsystem  TreatAsAtomicUnit=on  RTWFcnName=Iq_Fun
      settings: RTWFcnNameOpts=User specified
  Park : mcbeeMathTransformLib/Clarke to Park Angle Transform  AxisAlignment=D-axis  UseWithEmbedded=on  PhaseInput=Two inputs  ThetaInput=Electrical position  AngleInput=Radians  N_points=1024
      settings: LibrarySourceBlock=mcblib/Controls/Math Transforms/Park Transform
  SVPWMG : Subsystem  TreatAsAtomicUnit=on  RTWFcnName=SVPWM_Gen_Fun
      settings: RTWFcnNameOpts=User specified
  Unused_SatFlag : Terminator
  Unused_Sector : Terminator
  dq_voltage_limiter : Subsystem
  duty_u_cmd : Outport
  duty_v_cmd : Outport  Port=2
  duty_w_cmd : Outport  Port=3
  wires:
  [awq] -> Iq/5(du_q_z)
  [awd] -> Id/5(du_d_z)
  [we] -> Iq/4(we)
  [we] -> Id/4(we)
  [iq] -> Iq/3(iq)
  [iq] -> Id/3(iq)
  [id] -> Iq/2(id)
  [id] -> Id/2(id)
  iq_ref/1 -> Iq/1(Iq_ref)
  Id/1(ud_raw) -> dq_voltage_limiter/1(ud_raw)
  Iq/1(uq_raw) -> dq_voltage_limiter/2(uq_raw)
  PI_Reset_EN/1 -> [reset]
  id_ref/1 -> Id/1(id_ref)
  [reset] -> Id/6(PI_Reset_EN)
  [reset] -> Iq/6(PI_Reset_EN)
  InversePark/2 -> SVPWMG/2(Vbeta)
  InversePark/1 -> SVPWMG/1(Valpha)
  dq_voltage_limiter/2(uq_lim) -> InversePark/2  "uq"
  dq_voltage_limiter/1(ud_lim) -> InversePark/1  "ud"
  dq_voltage_limiter/5(sat_flag_z) -> Unused_SatFlag/1
  dq_voltage_limiter/4(du_q_z) -> [awq]
  dq_voltage_limiter/3(du_d_z) -> [awd]
  omega_e/1 -> [we]
  Park/2 -> [iq]
  Park/1 -> [id]
  theta_e/1 -> [theta]
  Clark/2(ibeta) -> Park/2
  Clark/1(ialpha) -> Park/1
  [theta] -> Park/3
  [theta] -> InversePark/3
  ia/1 -> Clark/1(ia)
  ib/1 -> Clark/2(ib)
  ic/1 -> Clark/3(ic)
  SVPWMG/1(duty_u_cmd) -> duty_u_cmd/1
  SVPWMG/2(duty_v_cmd) -> duty_v_cmd/1
  SVPWMG/3(duty_w_cmd) -> duty_w_cmd/1
  SVPWMG/4("N ") -> Unused_Sector/1

== system AXU5EV_R5_Reference/Motion_Control/FOC_Implementation/Float/FOC_Algorithm/Clark ==
  note: alpha=(A-0.5*(B+C))*2/3
      | Beta=sqrt(3)/2*(B-C)*2/3
  ia : Inport
  ib : Inport  Port=2
  ic : Inport  Port=3
  Add : Sum  Inputs=+--
  Add1 : Sum  Inputs=+-
  Gain : Gain  Gain=0.5
  Gain1 : Gain  Gain=0.5
  Gain2 : Gain  Gain=2/3
  Gain3 : Gain  Gain=1/sqrt(3)
  ialpha : Outport
  ibeta : Outport  Port=2
  wires:
  Gain1/1 -> Add/3
  ia/1 -> Add/1
  ib/1 -> Add1/1, Gain/1
  Add1/1 -> Gain3/1
  ic/1 -> Add1/2, Gain1/1
  Gain3/1 -> ibeta/1  "ibeta"
  Add/1 -> Gain2/1
  Gain2/1 -> ialpha/1  "ialf"
  Gain/1 -> Add/2

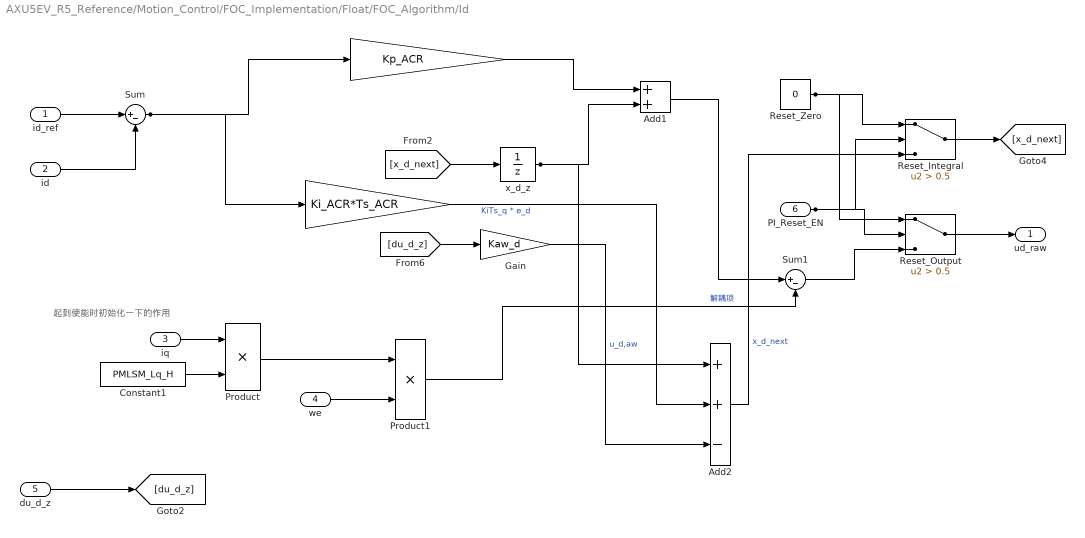
== system AXU5EV_R5_Reference/Motion_Control/FOC_Implementation/Float/FOC_Algorithm/Id ==
  note: 起到使能时初始化一下的作用
  id_ref : Inport
  id : Inport  Port=2
  iq : Inport  Port=3
  we : Inport  Port=4
  du_d_z : Inport  Port=5
  PI_Reset_EN : Inport  Port=6
  " " : Gain  Gain=Ki_ACR*Ts_ACR
  "  " : Gain  Gain=Kp_ACR
  Add1 : Sum
  Add2 : Sum  Inputs=++-
  Constant1 : Constant  Value=PMLSM_Lq_H
  Gain : Gain  Gain=Kaw_d
  Product : Product
  Product1 : Product
  Reset_Integral : Switch  Criteria=u2 > Threshold  Threshold=0.5  SaturateOnIntegerOverflow=off  InputSameDT=off
  Reset_Output : Switch  Criteria=u2 > Threshold  Threshold=0.5  SaturateOnIntegerOverflow=off  InputSameDT=off
  Reset_Zero : Constant  Value=0
  Sum : Sum  Inputs=|+-
  Sum1 : Sum  Inputs=|+-
  x_d_z : UnitDelay  SampleTime=-1
  ud_raw : Outport
  wires:
  Product1/1 -> Sum1/2  "解耦项"
  Add1/1 -> Sum1/1
  x_d_z/1 -> Add1/2, Add2/1
  Gain/1 -> Add2/3  "u_d,aw"
  " "/1 -> Add2/2  "KiTs_q * e_d"
  Sum1/1 -> Reset_Output/3
  Add2/1 -> Reset_Integral/3  "x_d_next"
  Reset_Zero/1 -> Reset_Integral/1, Reset_Output/1
  PI_Reset_EN/1 -> Reset_Integral/2, Reset_Output/2
  Reset_Integral/1 -> [x_d_next]
  Reset_Output/1 -> ud_raw/1
  iq/1 -> Product/1
  id_ref/1 -> Sum/1
  id/1 -> Sum/2
  Sum/1 -> " "/1, "  "/1
  we/1 -> Product1/2
  Product/1 -> Product1/1
  Constant1/1 -> Product/2
  "  "/1 -> Add1/1
  du_d_z/1 -> [du_d_z]
  [x_d_next] -> x_d_z/1
  [du_d_z] -> Gain/1

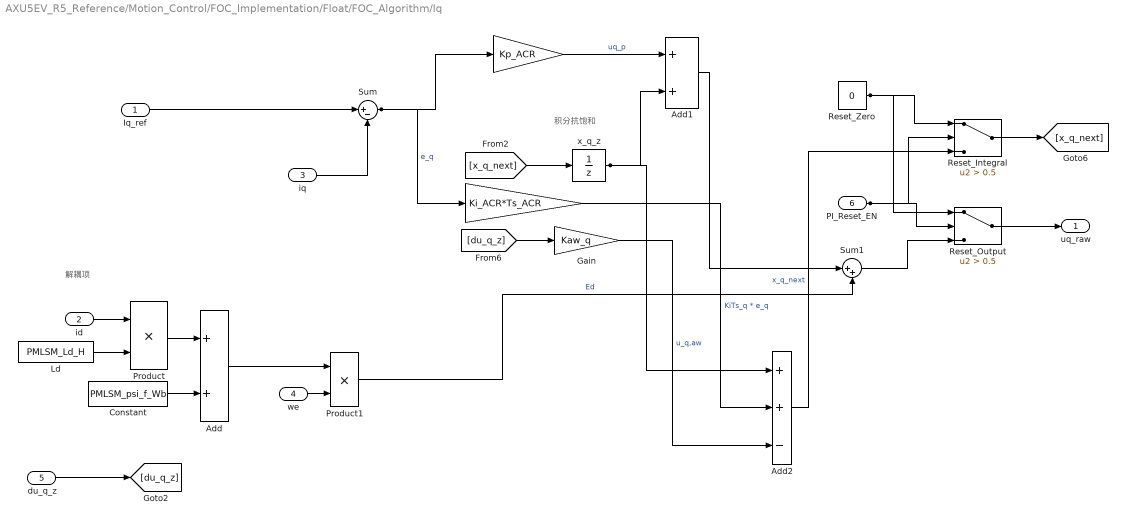
== system AXU5EV_R5_Reference/Motion_Control/FOC_Implementation/Float/FOC_Algorithm/Iq ==
  note: 解耦项
  note: 积分抗饱和
  Iq_ref : Inport
  id : Inport  Port=2
  iq : Inport  Port=3
  we : Inport  Port=4
  du_q_z : Inport  Port=5
  PI_Reset_EN : Inport  Port=6
  " " : Gain  Gain=Ki_ACR*Ts_ACR
  "  " : Gain  Gain=Kp_ACR
  Add : Sum
  Add1 : Sum
  Add2 : Sum  Inputs=++-
  Constant : Constant  Value=PMLSM_psi_f_Wb
  Gain : Gain  Gain=Kaw_q
  Ld : Constant  Value=PMLSM_Ld_H
  Product : Product
  Product1 : Product
  Reset_Integral : Switch  Criteria=u2 > Threshold  Threshold=0.5  SaturateOnIntegerOverflow=off  InputSameDT=off
  Reset_Output : Switch  Criteria=u2 > Threshold  Threshold=0.5  SaturateOnIntegerOverflow=off  InputSameDT=off
  Reset_Zero : Constant  Value=0
  Sum : Sum  Inputs=|+-
  Sum1 : Sum  Inputs=|++
  x_q_z : UnitDelay  SampleTime=-1
  uq_raw : Outport
  wires:
  Product1/1 -> Sum1/2  "Ed"
  Add1/1 -> Sum1/1
  Gain/1 -> Add2/3  "u_q,aw"
  " "/1 -> Add2/2  "KiTs_q * e_q"
  x_q_z/1 -> Add1/2, Add2/1
  Sum1/1 -> Reset_Output/3
  Add2/1 -> Reset_Integral/3  "x_q_next"
  Reset_Zero/1 -> Reset_Integral/1, Reset_Output/1
  PI_Reset_EN/1 -> Reset_Integral/2, Reset_Output/2
  Reset_Integral/1 -> [x_q_next]
  Reset_Output/1 -> uq_raw/1
  we/1 -> Product1/2
  iq/1 -> Sum/2
  id/1 -> Product/1
  Ld/1 -> Product/2
  Product/1 -> Add/1
  Constant/1 -> Add/2
  Add/1 -> Product1/1
  Sum/1 -> "  "/1, " "/1  "e_q"
  "  "/1 -> Add1/1  "uq_p"
  du_q_z/1 -> [du_q_z]
  [du_q_z] -> Gain/1
  [x_q_next] -> x_q_z/1
  Iq_ref/1 -> Sum/1

== system AXU5EV_R5_Reference/Motion_Control/FOC_Implementation/Float/FOC_Algorithm/SVPWMG ==
  Valpha : Inport
  Vbeta : Inport  Port=2
  Duty Calculate : Subsystem  TreatAsAtomicUnit=on  RTWFcnName=Duty_Caculate_Fun
      settings: RTWFcnNameOpts=User specified
  Sector Caculate : Subsystem  TreatAsAtomicUnit=on  RTWFcnName=Sector_Caculate_Fun
      settings: RTWFcnNameOpts=User specified
  T1T2 Calculate : Subsystem  TreatAsAtomicUnit=on  RTWFcnName=T1T2Caculate_Fun
      settings: RTWFcnNameOpts=User specified
  Udc : Constant  Value=Udc
  XYZ Calculate : Subsystem  TreatAsAtomicUnit=on  RTWFcnName=XYZ_Caculate_Fun
      settings: RTWFcnNameOpts=User specified
  duty_u_cmd : Outport
  duty_v_cmd : Outport  Port=2
  duty_w_cmd : Outport  Port=3
  "N " : Outport  Port=4
  wires:
  Vbeta/1 -> Sector Caculate/2(Ubeta), XYZ Calculate/2(Ubeta)
  T1T2 Calculate/1(T1) -> Duty Calculate/2(T1)
  Valpha/1 -> Sector Caculate/1(Ualpha), XYZ Calculate/1(Ualpha)
  T1T2 Calculate/2(T2) -> Duty Calculate/3(T2)
  Sector Caculate/1("N ") -> "N "/1, Duty Calculate/1(N), T1T2 Calculate/1(N)
  Udc/1 -> XYZ Calculate/3(Udc)
  XYZ Calculate/1(X) -> T1T2 Calculate/2(X)
  XYZ Calculate/2(Y) -> T1T2 Calculate/3(Y)
  XYZ Calculate/3(Z) -> T1T2 Calculate/4(Z)
  Duty Calculate/1(Duty_U) -> duty_u_cmd/1
  Duty Calculate/2(Duty_V) -> duty_v_cmd/1
  Duty Calculate/3(Duty_W) -> duty_w_cmd/1

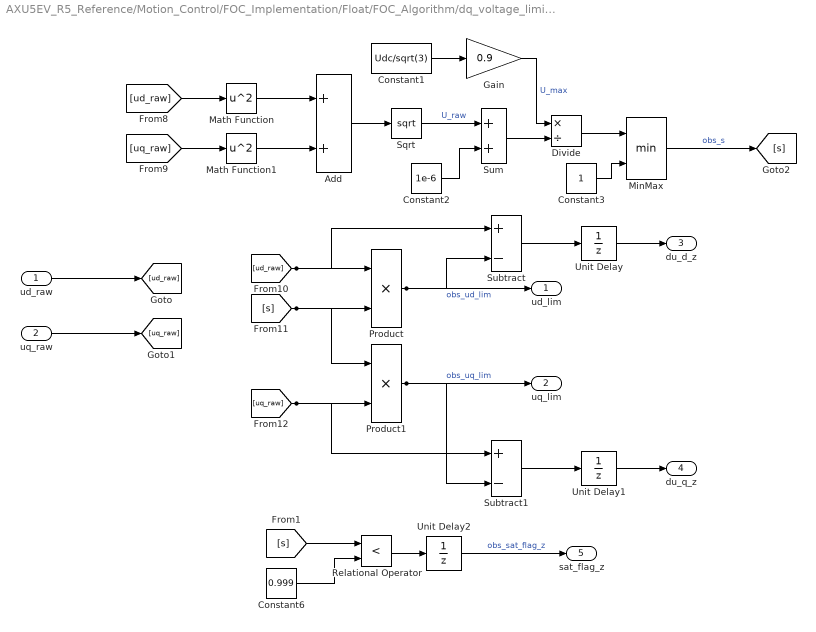
== system AXU5EV_R5_Reference/Motion_Control/FOC_Implementation/Float/FOC_Algorithm/dq_voltage_limiter ==
  ud_raw : Inport
  uq_raw : Inport  Port=2
  Add : Sum
  Constant1 : Constant  Value=Udc/sqrt(3)  OutDataTypeStr=double
  Constant2 : Constant  Value=1e-6  OutDataTypeStr=double
  Constant3 : Constant  OutDataTypeStr=double
  Constant6 : Constant  Value=0.999
  Divide : Product  Inputs=*/  OutDataTypeStr=double
  Gain : Gain  Gain=0.9  OutDataTypeStr=double
  Math Function : Math  Operator=square
  Math Function1 : Math  Operator=square
  MinMax : MinMax  Inputs=2
  Product : Product
  Product1 : Product  OutDataTypeStr=double
  Relational Operator : RelationalOperator  Operator=<  OutDataTypeStr=boolean  RndMeth=Simplest  InputSameDT=off
  Sqrt : Sqrt
  Subtract : Sum  Inputs=+-
  Subtract1 : Sum  Inputs=+-
  Sum : Sum
  Unit Delay : UnitDelay  SampleTime=-1
  Unit Delay1 : UnitDelay  SampleTime=-1
  Unit Delay2 : UnitDelay  SampleTime=-1
  ud_lim : Outport
  uq_lim : Outport  Port=2
  du_d_z : Outport  Port=3
  du_q_z : Outport  Port=4
  sat_flag_z : Outport  Port=5
  wires:
  Sum/1 -> Divide/2
  Constant2/1 -> Sum/2
  Constant3/1 -> MinMax/2
  Add/1 -> Sqrt/1
  Constant1/1 -> Gain/1
  Divide/1 -> MinMax/1
  Gain/1 -> Divide/1  "U_max"
  Sqrt/1 -> Sum/1  "U_raw"
  Math Function1/1 -> Add/2
  Math Function/1 -> Add/1
  [uq_raw] -> Math Function1/1
  [ud_raw] -> Math Function/1
  MinMax/1 -> [s]  "obs_s"
  Product1/1 -> uq_lim/1, Subtract1/2  "obs_uq_lim"
  [s] -> Product1/1, Product/2
  [ud_raw] -> Subtract/1, Product/1
  Product/1 -> Subtract/2, ud_lim/1  "obs_ud_lim"
  [uq_raw] -> Subtract1/1, Product1/2
  Subtract/1 -> Unit Delay/1
  Subtract1/1 -> Unit Delay1/1
  ud_raw/1 -> [ud_raw]
  uq_raw/1 -> [uq_raw]
  Unit Delay/1 -> du_d_z/1
  Unit Delay1/1 -> du_q_z/1
  Constant6/1 -> Relational Operator/2
  [s] -> Relational Operator/1
  Relational Operator/1 -> Unit Delay2/1
  Unit Delay2/1 -> sat_flag_z/1  "obs_sat_flag_z"

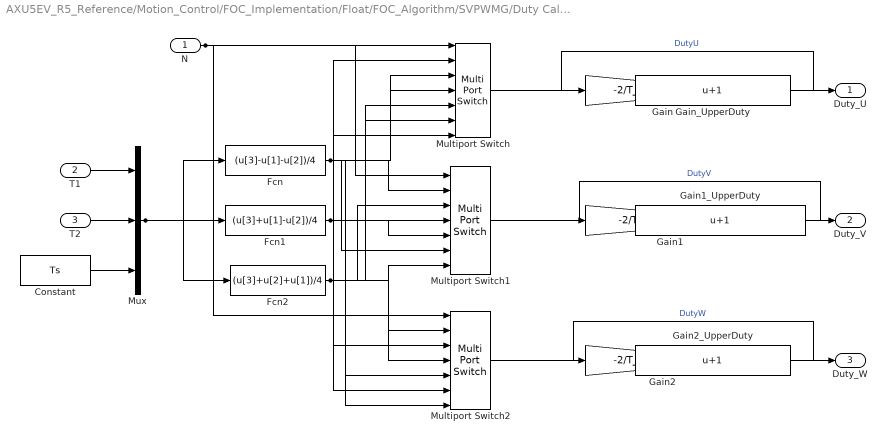
== system AXU5EV_R5_Reference/Motion_Control/FOC_Implementation/Float/FOC_Algorithm/SVPWMG/Duty Calculate ==
  N : Inport
  T1 : Inport  Port=2
  T2 : Inport  Port=3
  Constant : Constant  Value=Ts
  Fcn : Fcn  Expr=(u[3]-u[1]-u[2])/4
  Fcn1 : Fcn  Expr=(u[3]+u[1]-u[2])/4
  Fcn2 : Fcn  Expr=(u[3]+u[2]+u[1])/4
  Gain : Gain  Gain=-2/T_pwm
  Gain1 : Gain  Gain=-2/T_pwm
  Gain1_UpperDuty : Bias  Bias=1  SaturateOnIntegerOverflow=off
  Gain2 : Gain  Gain=-2/T_pwm
  Gain2_UpperDuty : Bias  Bias=1  SaturateOnIntegerOverflow=off
  Gain_UpperDuty : Bias  Bias=1  SaturateOnIntegerOverflow=off
  Multiport Switch : MultiPortSwitch  Inputs=6  SaturateOnIntegerOverflow=off  InputSameDT=off
  Multiport Switch1 : MultiPortSwitch  Inputs=6  SaturateOnIntegerOverflow=off  InputSameDT=off
  Multiport Switch2 : MultiPortSwitch  Inputs=6  SaturateOnIntegerOverflow=off  InputSameDT=off
  Mux : Mux  Inputs=3
  Duty_U : Outport
  Duty_V : Outport  Port=2
  Duty_W : Outport  Port=3
  wires:
  Gain2_UpperDuty/1 -> Duty_W/1
  Gain2/1 -> Gain2_UpperDuty/1  "DutyW"
  Gain1_UpperDuty/1 -> Duty_V/1
  Gain1/1 -> Gain1_UpperDuty/1  "DutyV"
  Gain_UpperDuty/1 -> Duty_U/1
  Gain/1 -> Gain_UpperDuty/1  "DutyU"
  Mux/1 -> Fcn2/1, Fcn/1, Fcn1/1
  Constant/1 -> Mux/3
  T2/1 -> Mux/2
  T1/1 -> Mux/1
  Multiport Switch2/1 -> Gain2/1
  Multiport Switch1/1 -> Gain1/1
  Multiport Switch/1 -> Gain/1
  Fcn/1 -> Multiport Switch/3, Multiport Switch/4, Multiport Switch1/6, Multiport Switch2/5, Multiport Switch2/7, Multiport Switch1/2
  Fcn1/1 -> Multiport Switch1/5, Multiport Switch2/3, Multiport Switch2/6, Multiport Switch1/4, Multiport Switch/7, Multiport Switch/2
  Fcn2/1 -> Multiport Switch/5, Multiport Switch/6, Multiport Switch1/3, Multiport Switch1/7, Multiport Switch2/2, Multiport Switch2/4
  N/1 -> Multiport Switch2/1, Multiport Switch1/1, Multiport Switch/1

== system AXU5EV_R5_Reference/Motion_Control/FOC_Implementation/Float/FOC_Algorithm/SVPWMG/Sector Caculate ==
  Ualpha : Inport
  Ubeta : Inport  Port=2
  B0 : Fcn  Expr=u[2]
  B1 : Fcn  Expr=u[1]*0.866-0.5*u[2]
  B2 : Fcn  Expr=-u[1]*0.866-u[2]*0.5
  Constant : Constant
  Constant1 : Constant  Value=0
  Mux : Mux  Inputs=2
  Mux1 : Mux  Inputs=3
  N : Fcn  Expr=4*u[3]+2*u[2]+u[1]
  Switch : Switch  Criteria=u2 > Threshold  SaturateOnIntegerOverflow=off  InputSameDT=off
  Switch1 : Switch  SaturateOnIntegerOverflow=off  InputSameDT=off
  Switch2 : Switch  Criteria=u2 > Threshold  SaturateOnIntegerOverflow=off  InputSameDT=off
  "N " : Outport  VectorParamsAs1DForOutWhenUnconnected=off
  wires:
  Switch2/1 -> Mux1/3
  Switch/1 -> Mux1/1
  Ualpha/1 -> Mux/1
  Ubeta/1 -> Mux/2
  Mux/1 -> B2/1, B1/1, B0/1
  B0/1 -> Switch/2
  B1/1 -> Switch1/2
  B2/1 -> Switch2/2
  Constant/1 -> Switch/1, Switch2/1, Switch1/1
  Constant1/1 -> Switch/3, Switch1/3, Switch2/3
  Switch1/1 -> Mux1/2
  Mux1/1 -> N/1
  N/1 -> "N "/1  "N"

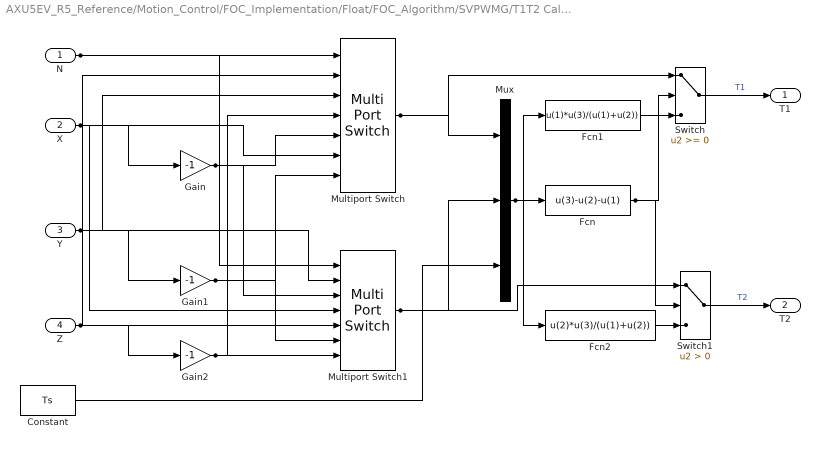
== system AXU5EV_R5_Reference/Motion_Control/FOC_Implementation/Float/FOC_Algorithm/SVPWMG/T1T2 Calculate ==
  N : Inport
  X : Inport  Port=2
  Y : Inport  Port=3
  Z : Inport  Port=4
  Constant : Constant  Value=Ts
  Fcn : Fcn  Expr=u(3)-u(2)-u(1)
  Fcn1 : Fcn  Expr=u(1)*u(3)/(u(1)+u(2))
  Fcn2 : Fcn  Expr=u(2)*u(3)/(u(1)+u(2))
  Gain : Gain  Gain=-1
  Gain1 : Gain  Gain=-1
  Gain2 : Gain  Gain=-1
  Multiport Switch : MultiPortSwitch  Inputs=6  SaturateOnIntegerOverflow=off  InputSameDT=off
  Multiport Switch1 : MultiPortSwitch  Inputs=6  SaturateOnIntegerOverflow=off  InputSameDT=off
  Mux : Mux  Inputs=3
  Switch : Switch  SaturateOnIntegerOverflow=off  InputSameDT=off
  Switch1 : Switch  Criteria=u2 > Threshold  SaturateOnIntegerOverflow=off  InputSameDT=off
  T1 : Outport  VectorParamsAs1DForOutWhenUnconnected=off
  T2 : Outport  Port=2  VectorParamsAs1DForOutWhenUnconnected=off
  wires:
  Constant/1 -> Mux/3
  Switch1/1 -> T2/1  "T2"
  Switch/1 -> T1/1  "T1"
  Fcn2/1 -> Switch1/3
  Fcn1/1 -> Switch/3
  Fcn/1 -> Switch/2, Switch1/2
  Mux/1 -> Fcn1/1, Fcn/1, Fcn2/1
  Multiport Switch/1 -> Switch/1, Mux/1
  Multiport Switch1/1 -> Switch1/1, Mux/2
  N/1 -> Multiport Switch/1, Multiport Switch1/1
  Y/1 -> Multiport Switch/3, Multiport Switch1/2, Gain1/1
  Z/1 -> Multiport Switch1/5, Multiport Switch/2, Gain2/1
  X/1 -> Gain/1, Multiport Switch/6, Multiport Switch1/4
  Gain/1 -> Multiport Switch1/3, Multiport Switch/5
  Gain2/1 -> Multiport Switch/4, Multiport Switch1/7
  Gain1/1 -> Multiport Switch1/6, Multiport Switch/7

== system AXU5EV_R5_Reference/Motion_Control/FOC_Implementation/Float/FOC_Algorithm/SVPWMG/XYZ Calculate ==
  Ualpha : Inport
  Ubeta : Inport  Port=2
  Udc : Inport  Port=3
  Add : Sum
  Add1 : Sum  Inputs=+-
  Constant1 : Constant  Value=Ts
  Gain : Gain  Gain=3/2
  Gain1 : Gain  Gain=1.7321
  Gain2 : Gain  Gain=0.866
  Math Function : Math  Operator=reciprocal
  Product{,1..3} (4 alike) : Product
  X : Outport
  Y : Outport  Port=2
  Z : Outport  Port=3
  wires:
  Ualpha/1 -> Gain/1
  Udc/1 -> Math Function/1
  Math Function/1 -> Product/2
  Ubeta/1 -> Gain2/1, Gain1/1
  Gain1/1 -> Product1/1
  Product/1 -> Product2/2, Product3/2, Product1/2
  Gain2/1 -> Add/1, Add1/1
  Gain/1 -> Add1/2, Add/2
  Product1/1 -> X/1  "X"
  Add/1 -> Product3/1
  Add1/1 -> Product2/1
  Product2/1 -> Z/1  "Z"
  Product3/1 -> Y/1  "Y"
  Constant1/1 -> Product/1

== stateflow chart AXU5EV_R5_Reference/Alignment_Task/Enabled_Original_MIL/Angle_Init ==
  state IDLE
    entry:
    Angle_Init_EN   = 0;
    Init_Done       = 0;
    id_init_ref     = 0;
    Init_State_Num  = 0;
  note: 固定电角度，缓慢建立 d 轴电流。
  note: 保持固定电角度，让动子吸附稳定。
  state RAMP_ID
    entry:
    Angle_Init_EN   = 1;
    Init_Done       = 0;
    id_init_ref     = 0;
    Init_State_Num  = 1;
    during:
    Angle_Init_EN = 1;
    Init_Done     = 0;
    id_init_ref = id_init_ref + Id_Init_Step;
    if (id_init_ref > Id_Init_Target)
    id_init_ref = Id_Init_Target;
    end
  state HOLD_ALIGN
    entry:
    Angle_Init_EN   = 1;
    Init_Done       = 0;
    id_init_ref     = Id_Init_Target;
    Init_State_Num  = 2;
    during:
    Angle_Init_EN = 1;
    Init_Done     = 0;
    id_init_ref   = Id_Init_Target;
  state RAMP_DOWN_ID
    entry:
    Angle_Init_EN   = 1;
    Init_Done       = 0;
    id_init_ref     = Id_Init_Target;
    Init_State_Num  = 3;
    during:
    Angle_Init_EN = 1;
    Init_Done     = 0;
    id_init_ref = id_init_ref - Id_Init_Target/Id_Release_Ramp_Ticks;
    if (id_init_ref < 0)
    id_init_ref = 0;
    end
    Theta_Offset_auto = theta_offset_mem;
  state DONE
    entry:
    Angle_Init_EN   = 0;
    Init_Done       = 1;
    id_init_ref     = 0;
    Init_State_Num  = 4;
    during:
    Angle_Init_EN = 0;
    Init_Done = 1;
    id_init_ref = 0;
    Init_State_Num = 4;
    Theta_Offset_auto = theta_offset_mem;
  HOLD_ALIGN -> IDLE [order 1] : [Init_Reset > 0.5 || travel_fault_latch > 0.5]
  RAMP_ID -> IDLE [order 1] : [Init_Reset > 0.5 || travel_fault_latch > 0.5]
  (default) -> IDLE
  IDLE -> RAMP_ID : [Init_Start > 0.5 && Init_Reset < 0.5 && travel_fault_latch < 0.5]
  RAMP_ID -> HOLD_ALIGN [order 2] : [after(Ramp_Ticks, tick)]
  RAMP_DOWN_ID -> IDLE [order 2] : [Init_Reset > 0.5 || travel_fault_latch > 0.5]
  DONE -> IDLE : [Init_Reset > 0.5 || travel_fault_latch > 0.5]
  HOLD_ALIGN -> RAMP_DOWN_ID [order 2] : [after(Hold_Ticks, tick)]
      | {x_align_mm_latch = x_mm;
      | theta_offset_mem = mod(theta_align_const - 2*pi*x_align_mm_latch/Tau_e_mm, 2*pi);
      | Theta_Offset_auto = theta_offset_mem;}
  RAMP_DOWN_ID -> DONE [order 1] : [after(Id_Release_Ramp_Ticks, tick)]
  data: Init_Start input; Init_Reset input; travel_fault_latch input; Init_Done output; Init_State_Num output; theta_align_const parameter; Tau_e_mm parameter; Id_Init_Target parameter; Ramp_Ticks parameter; Hold_Ticks parameter; Id_Init_Step parameter; id_init_ref output; Angle_Init_EN output; x_mm input; Theta_Offset_auto output; x_align_mm_latch output; theta_offset_mem local; Id_Release_Ramp_Ticks parameter
